simulink model "meteorprocess_model6"  (R2025b)
settings: Solver=VariableStepAuto  StartTime=0.0  StopTime=30  RelTol=1e-3
undefined symbols (not defined in the file or in its folder): designMultirateFIR
libraries: dsparch4 x2, dspmlti4 x1, dspvision x1
settings Model: Creator=bruce  LastModifiedBy=bruce
settings OptimizationCC: ReuseModelBlockBuffer=off
settings RTWCC: GPUComputeCapability=3.5

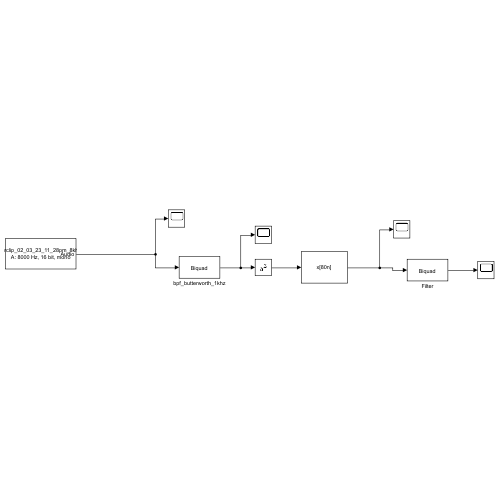
[thumbnail: Simulink's stored preview of the top-level diagram]
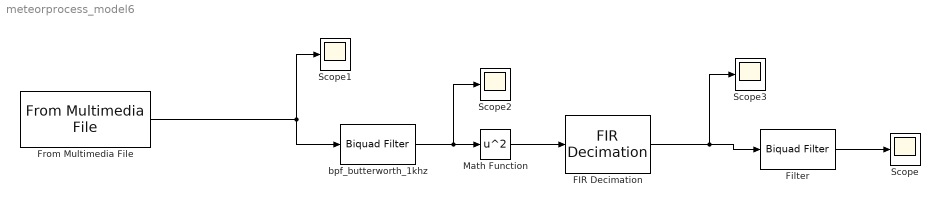
== system meteorprocess_model6 ==
  FIR Decimation : dspmlti4/FIR Decimation  FilterSource=Auto  h=designMultirateFIR(1,2)  D=80  filtStruct=Direct form  FilterObject=FDECIM  InputProcessing=Columns as channels (frame based)  framing=Allow multirate processing  AllowArbitraryInputLength=off  inputOffset=0  outputBufInitCond=0  roundingMode=Floor  overflowMode=off  firstCoeffDataTypeStr=Inherit: Same word length as input  firstCoeffMin=[]  firstCoeffMax=[]  firstCoeffLastDataTypeStr=Inherit: Same word length as input  outputDataTypeStr=Inherit: Same as accumulator  outputMin=[]  outputMax=[]  outputLastDataTypeStr=Inherit: Same as accumulator
  Filter : dsparch4/Biquad Filter  Tag=BlockMethodSubSystem  FilterSource=Dialog parameters  CoeffSource=Specify via dialog  FilterObject=BQF  IIRFiltStruct=Direct form II  BiQuadCoeffs=[1 2 1 1 -1.14298050253990113 0.412801598096188771]  ScaleValues=[0.0674552738890718956;1]  IC=0  ICnum=0  ICden=0  a0Flag=Warning  optimizeScaleValues=on  ScaleValueMode=Specify via input port (g)  InputProcessing=Columns as channels (frame based)  roundingMode=Floor  overflowMode=off  scaleValueFracLength=14  denProdOutputFracLength=30  denAccumFracLength=30  secondMemoryFracLength=15
  From Multimedia File : dspvision/From Multimedia File  inputFilename=C:\Users\bruce\Documents\MATLAB\meteoraudio\meteorclip_02_03_23_11_28pm_8khz.wav  readRange=[1 Inf]  loop=on  numPlays=inf  outputStreams=Audio only  videoDataType=single  audioDataType=double  inheritSampleTime=on  userDefinedSampleTime=1/30  noAudioOutput=off  isIntensityVideo=off  fourcc=RGB  colorVideoFormat=Separate color signals  outputEOF=off  dataOrg=Column-major  audioFrameSize=1  computeAudioFrameSize=off  outSamplingMode=Sample based
      settings: LibrarySourceBlock=audiosources/From Multimedia File
  Math Function : Math  Operator=square
  Scope{,1..3} (4 alike) : Scope
      Scope settings: ActiveDisplayYMinimum=-0.0058981818415032652  ActiveDisplayYMaximum=0.029934942408496697
      Scope1 settings: ActiveDisplayYMinimum=-0.70763411926472708  ActiveDisplayYMaximum=0.63637540454479669
      Scope2 settings: ActiveDisplayYMinimum=-0.47418104762596291  ActiveDisplayYMaximum=0.47689900955893777  DataLoggingVariableName=ScopeData2
      Scope3 settings: ActiveDisplayYMinimum=-0.00673  ActiveDisplayYMaximum=0.04763  DataLoggingVariableName=ScopeData3
  bpf_butterworth_1khz : dsparch4/Biquad Filter  Tag=BlockMethodSubSystem  FilterSource=Dialog parameters  CoeffSource=Specify via dialog  FilterObject=BQF  IIRFiltStruct=Direct form II  BiQuadCoeffs=[1 0 -1 1 -1.2615688871702464 0.889316102872194425;1 0 -1 1 -1.41858929976926107 0.900470197356578517]  ScaleValues=[0.0744494271991443801;0.0744494271991443801;1]  IC=0  ICnum=0  ICden=0  a0Flag=Warning  optimizeScaleValues=on  ScaleValueMode=Specify via input port (g)  roundingMode=Floor  overflowMode=off  scaleValueFracLength=14  denProdOutputFracLength=30  denAccumFracLength=30  secondMemoryFracLength=15
  wires:
  bpf_butterworth_1khz/1 -> Scope2/1, Math Function/1
  From Multimedia File/1 -> bpf_butterworth_1khz/1, Scope1/1
  Math Function/1 -> FIR Decimation/1
  Filter/1 -> Scope/1
  FIR Decimation/1 -> Filter/1, Scope3/1
